simulink model "ACB_RealTime_Simulation"  (R2024b)
settings: Solver=VariableStepAuto  StartTime=0.0  StopTime=10.0  RelTol=1e-3
settings Model: Creator=Grishma  LastModifiedBy=Grishma

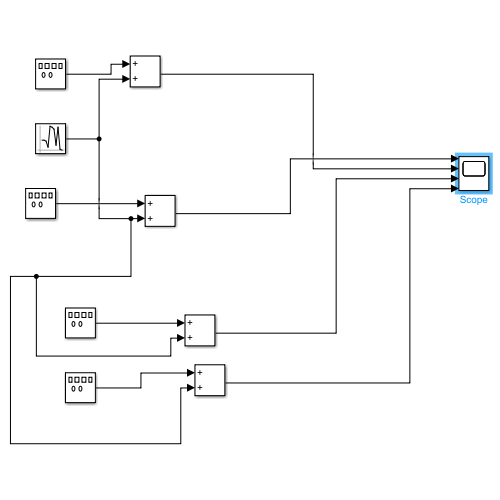
[thumbnail: Simulink's stored preview of the top-level diagram]
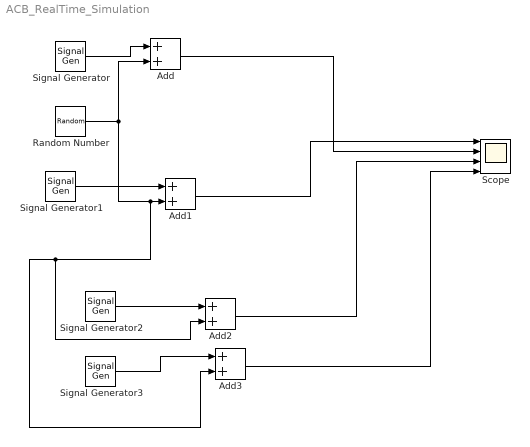
== system ACB_RealTime_Simulation ==
  Add{,1..3} (4 alike) : Sum
  Random Number : RandomNumber  Mean=0.05  SampleTime=0.1
  Scope : Scope  NumInputPorts=4
  Signal Generator : SignalGenerator  Amplitude=50  Frequency=5  Units=rad/sec
  Signal Generator1 : SignalGenerator  Amplitude=52  Frequency=5  Units=rad/sec
  Signal Generator2 : SignalGenerator  Amplitude=55  Frequency=5  Units=rad/sec
  Signal Generator3 : SignalGenerator  Amplitude=58  Frequency=5  Units=rad/sec
  wires:
  Random Number/1 -> Add2/2, Add3/2, Add1/2, Add/2
  Signal Generator/1 -> Add/1
  Signal Generator1/1 -> Add1/1
  Signal Generator2/1 -> Add2/1
  Signal Generator3/1 -> Add3/1
  Add/1 -> Scope/2
  Add1/1 -> Scope/1
  Add2/1 -> Scope/3
  Add3/1 -> Scope/4
